simulink model "INS"  (R2018b)
settings: configuration reference "ins_config" (kept outside this file)
values from neighbouring files (symbols this model uses):
  INS_EXPORT = Simulink.Parameter(INS_EXPORT_VALUE)    [ins_model_init.m]
  INS_PARAM = Simulink.Parameter(INS_PARAM_VALUE)    [ins_model_init.m]
undefined symbols (not defined in the file or in its folder): DiscIntNeverNeededParam, INS_CONST, INS_EXPORT_VALUE, Sensor_Meas
libraries: simulink x131, FMT_Model_Lib x48
(part 3 of 6)

== system INS/Data_Fusion/Rotation_Filter/AHRS/Correct/Gyro_Bias_Correction ==
  att_B_correction : Inport
  IMU_Data : Inport  Port=2
  Abs : Abs
  Bus Selector : BusSelector  OutputSignals=acc_B_mPs2
  Compare To Constant : simulink/Logic and Bit Operations/Compare To Constant  relop=<=  const=1  OutDataTypeStr=boolean
  Constant : Constant  Value=INS_CONST.g  OutDataTypeStr=single
  Data Type Conversion : DataTypeConversion  OutDataTypeStr=single
  Demux : Demux  Outputs=3
  Gain1 : Gain  Gain=INS_PARAM.BIAS_G_GAIN
  Gain2 : Gain  Gain=INS_PARAM.BIAS_G_GAIN
  Gain3 : Gain  Gain=0
  MX Product1 : Product  RndMeth=Simplest
  Mux : Mux  Inputs=3
  Saturation2 : Saturate  UpperLimit=0.1/180*pi  LowerLimit=-0.1/180*pi
  Second Order LPF : FMT_Model_Lib/Filter/Second Order LPF  fc=5  zeta=0.707
      settings: SourceProductName=FMT Toolbox
  Subtract : Sum  Inputs=+-
  Vector Modulus : FMT_Model_Lib/Math/Vector Modulus
      settings: SourceProductName=FMT Toolbox
  bias_g_B_correction : Outport
  wires:
  IMU_Data/1 -> Bus Selector/1
  Saturation2/1 -> bias_g_B_correction/1  "bias_g_correction"
  Compare To Constant/1 -> Data Type Conversion/1
  Bus Selector/1 -> Vector Modulus/1  "<acc_B_mPs2>"
  MX Product1/1 -> Second Order LPF/1
  att_B_correction/1 -> MX Product1/1
  Vector Modulus/1 -> Subtract/1
  Mux/1 -> Saturation2/1
  Constant/1 -> Subtract/2
  Subtract/1 -> Abs/1
  Abs/1 -> Compare To Constant/1
  Data Type Conversion/1 -> MX Product1/2
  Second Order LPF/1 -> Demux/1
  Demux/1 -> Gain1/1
  Demux/2 -> Gain2/1
  Demux/3 -> Gain3/1
  Gain1/1 -> Mux/1
  Gain2/1 -> Mux/2
  Gain3/1 -> Mux/3

== system INS/Data_Fusion/Rotation_Filter/AHRS/Update/Attitude_Update ==
  att_reset : Inport
  quat_0 : Inport  Port=2
  att_B_correction : Inport  Port=3
  Constant : Constant  Value=0  OutDataTypeStr=single
  Delay1 : Delay  DelayLength=1  InitialConditionSource=Input port  InitialCondition=[1.0 0 0 0]
      settings: InputPortMap=u0,p4
  Gain1 : Gain  Gain=0.5  OutMin=-450*pi/180  OutMax=450*pi/180  RndMeth=Simplest
  Mux1 : Mux  Inputs=2
  Quaternion Multiply1 : FMT_Model_Lib/Quaternion/Quaternion Multiply
      settings: SourceProductName=FMT Toolbox
  Quaternion Normalize1 : FMT_Model_Lib/Quaternion/Quaternion Normalize
      settings: SourceProductName=FMT Toolbox
  Quaternion To DCM : FMT_Model_Lib/Quaternion/Quaternion To DCM
      settings: SourceProductName=FMT Toolbox
  Sum : Sum  Inputs=++|
  Switch : Switch  Criteria=u2 > Threshold
  Transpose : Math  Operator=transpose  SaturateOnIntegerOverflow=on
  dT : Gain  Gain=INS_CONST.dt  OutDataTypeStr=Inherit: Same as input
  att_quat : Outport
  DCM_OB : Outport  Port=2
  wires:
  att_reset/1 -> Switch/2
  quat_0/1 -> Switch/1, Delay1/2
  att_B_correction/1 -> Mux1/2
  Mux1/1 -> Quaternion Multiply1/2
  Constant/1 -> Mux1/1
  Quaternion To DCM/1 -> Transpose/1
  Transpose/1 -> DCM_OB/1
  Sum/1 -> Quaternion Normalize1/1
  dT/1 -> Sum/1
  Delay1/1 -> Quaternion Multiply1/1, Sum/2
  Quaternion Multiply1/1 -> Gain1/1
  Gain1/1 -> dT/1
  Switch/1 -> Delay1/1
  Quaternion Normalize1/1 -> att_quat/1, Switch/3, Quaternion To DCM/1

== system INS/Data_Fusion/Rotation_Filter/AHRS/Update/Attitude_Update1 ==
  att_reset : Inport
  quat_0 : Inport  Port=2
  att_B_correction : Inport  Port=3
  Constant : Constant  Value=0  OutDataTypeStr=single
  Discrete-Time Integrator : DiscreteIntegrator  ExternalReset=level  InitialConditionSource=external  SampleTime=-1  ICPrevOutput=DiscIntNeverNeededParam  ICPrevScaledInput=DiscIntNeverNeededParam
  Gain2 : Gain  Gain=0.5  OutMin=-450*pi/180  OutMax=450*pi/180  RndMeth=Simplest
  Mux1 : Mux  Inputs=2
  Quaternion Modulus : FMT_Model_Lib/Quaternion/Quaternion Modulus
      settings: SourceProductName=FMT Toolbox
  Quaternion Multiply : FMT_Model_Lib/Quaternion/Quaternion Multiply
      settings: SourceProductName=FMT Toolbox
  Quaternion Normalize : FMT_Model_Lib/Quaternion/Quaternion Normalize
      settings: SourceProductName=FMT Toolbox
  Quaternion To DCM : FMT_Model_Lib/Quaternion/Quaternion To DCM
      settings: SourceProductName=FMT Toolbox
  Transpose : Math  Operator=transpose  SaturateOnIntegerOverflow=on
  att_quat : Outport
  DCM_OB : Outport  Port=2
  wires:
  att_reset/1 -> Discrete-Time Integrator/2
  quat_0/1 -> Discrete-Time Integrator/3
  Gain2/1 -> Discrete-Time Integrator/1
  Quaternion Multiply/1 -> Gain2/1
  att_B_correction/1 -> Mux1/2
  Mux1/1 -> Quaternion Multiply/2
  Constant/1 -> Mux1/1
  Quaternion Normalize/1 -> Quaternion To DCM/1, Quaternion Multiply/1, att_quat/1
  Discrete-Time Integrator/1 -> Quaternion Modulus/1, Quaternion Normalize/1  "dd3"
  Quaternion To DCM/1 -> Transpose/1
  Transpose/1 -> DCM_OB/1
  Quaternion Modulus/1 -> ?  "dd4"

== system INS/Data_Fusion/Rotation_Filter/AHRS/Update/Gyro_Bias_Update ==
  bias_g_correction : Inport
  gyr_B_radPs : Inport  Port=2
  Discrete-Time Integrator2 : DiscreteIntegrator  SampleTime=-1  LimitOutput=on  UpperSaturationLimit=45/180*pi  LowerSaturationLimit=-45/180*pi  ICPrevOutput=DiscIntNeverNeededParam  ICPrevScaledInput=DiscIntNeverNeededParam
  Sum1 : Sum  Inputs=++|
  gyr_B_correction : Outport
  bias_g : Outport  Port=2
  wires:
  bias_g_correction/1 -> Discrete-Time Integrator2/1
  Sum1/1 -> gyr_B_correction/1
  Discrete-Time Integrator2/1 -> Sum1/1, bias_g/1
  gyr_B_radPs/1 -> Sum1/2

== system INS/Data_Fusion/Rotation_Filter/RF_Data_PreProcess/Attitude_Reset/sample_valid ==
  valid : Inport
  Add : Sum  AccumDataTypeStr=uint32
  Data Type Conversion : DataTypeConversion  OutDataTypeStr=uint32
  Delay : Delay  DelayLength=1
  Saturation : Saturate  UpperLimit=10000  LowerLimit=0
  valid_samples : simulink/Logic and Bit Operations/Compare To Constant  relop=>  const=50  OutDataTypeStr=boolean
  imu_valid : Outport
  wires:
  Add/1 -> Saturation/1
  valid_samples/1 -> imu_valid/1
  Delay/1 -> Add/2
  valid/1 -> Data Type Conversion/1
  Data Type Conversion/1 -> Add/1
  Saturation/1 -> valid_samples/1, Delay/1

== system INS/Data_Fusion/Rotation_Filter/RF_Data_PreProcess/Attitude_Reset/sample_valid1 ==
  valid : Inport
  Add : Sum  AccumDataTypeStr=uint32
  Data Type Conversion : DataTypeConversion  OutDataTypeStr=uint32
  Delay : Delay  DelayLength=1
  Saturation : Saturate  UpperLimit=10000  LowerLimit=0
  valid_samples : simulink/Logic and Bit Operations/Compare To Constant  relop=>  const=50  OutDataTypeStr=boolean
  mag_valid : Outport
  wires:
  Add/1 -> Saturation/1
  valid_samples/1 -> mag_valid/1
  Delay/1 -> Add/2
  valid/1 -> Data Type Conversion/1
  Data Type Conversion/1 -> Add/1
  Saturation/1 -> valid_samples/1, Delay/1

== system INS/Data_Fusion/Rotation_Filter/RF_Data_PreProcess/Initial_Attitude/Heading_Vector ==
  Sensor_Data : Inport
  Bus Selector1 : BusSelector  OutputSignals=Mag_Data.mag_norm_B
  Bus Selector2 : BusSelector  OutputSignals=GPS_Data.heading_valid,ExternalPos_Data.height_valid
  Bus Selector3 : BusSelector  OutputSignals=GPS_Data.heading_rad,ExternalPos_Data.psi
  Constant : Constant  Value=[1; 0; 0]  VectorParams1D=off  OutDataTypeStr=single
  Logical Operator : Logic  Operator=OR  AllPortsSameDT=off  OutDataTypeStr=boolean
  Multiply : Product  Multiplication=Matrix(*)
  Psi To DCM : FMT_Model_Lib/Transformation/Psi To DCM
      settings: SourceProductName=FMT Toolbox
  Switch : Switch  Criteria=u2 > Threshold
  Switch1 : Switch  Criteria=u2 > Threshold
  Vector Normalize : FMT_Model_Lib/Math/Vector Normalize
      settings: SourceProductName=FMT Toolbox
  heading_vec : Outport
  wires:
  Psi To DCM/1 -> Multiply/1
  Bus Selector1/1 -> Switch/3  "<mag_norm_B>"
  Switch/1 -> heading_vec/1
  Switch1/1 -> Psi To DCM/1  "<psi>"
  Logical Operator/1 -> Switch/2  "<heading_valid>"
  Sensor_Data/1 -> Bus Selector3/1, Bus Selector2/1, Bus Selector1/1
  Constant/1 -> Multiply/2
  Multiply/1 -> Vector Normalize/1
  Vector Normalize/1 -> Switch/1
  Bus Selector2/2 -> Logical Operator/2  "<height_valid>"
  Bus Selector2/1 -> Switch1/2, Logical Operator/1  "<heading_valid>"
  Bus Selector3/1 -> Switch1/1  "<heading_rad>"
  Bus Selector3/2 -> Switch1/3  "<psi>"

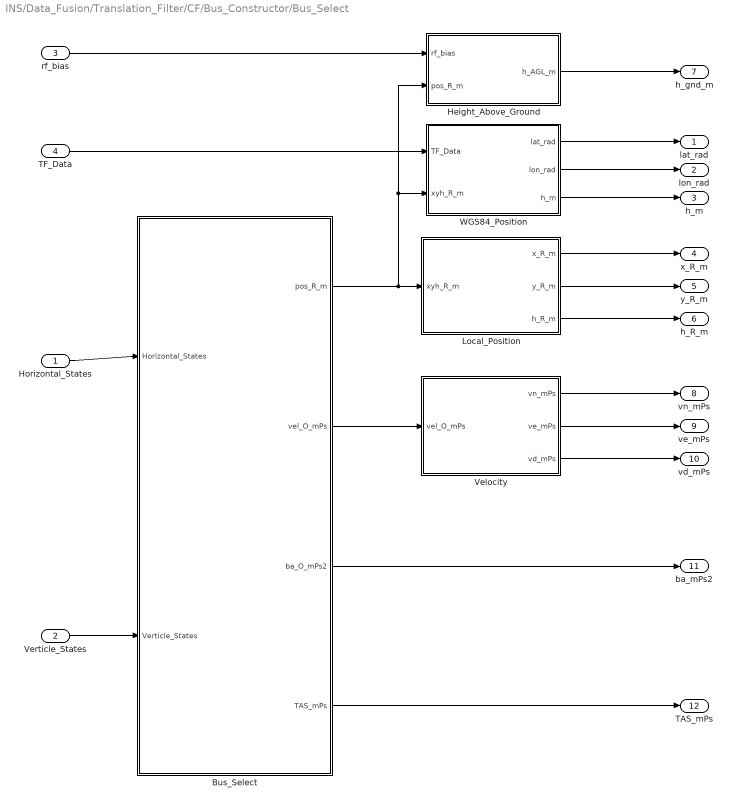
== system INS/Data_Fusion/Translation_Filter/CF/Bus_Constructor/Bus_Select ==
  Horizontal_States : Inport
  Verticle_States : Inport  Port=2
  rf_bias : Inport  Port=3
  TF_Data : Inport  Port=4
  Bus_Select : Subsystem
  Height_Above_Ground : Subsystem
  Local_Position : Subsystem
  Velocity : Subsystem
  WGS84_Position : Subsystem
  lat_rad : Outport
  lon_rad : Outport  Port=2
  h_m : Outport  Port=3
  x_R_m : Outport  Port=4
  y_R_m : Outport  Port=5
  h_R_m : Outport  Port=6
  h_gnd_m : Outport  Port=7
  vn_mPs : Outport  Port=8
  ve_mPs : Outport  Port=9
  vd_mPs : Outport  Port=10
  ba_mPs2 : Outport  Port=11
  TAS_mPs : Outport  Port=12
  wires:
  WGS84_Position/1(lat_rad) -> lat_rad/1
  TF_Data/1 -> WGS84_Position/1(TF_Data)
  WGS84_Position/2(lon_rad) -> lon_rad/1
  WGS84_Position/3(h_m) -> h_m/1
  Local_Position/1(x_R_m) -> x_R_m/1
  Local_Position/2(y_R_m) -> y_R_m/1
  Local_Position/3(h_R_m) -> h_R_m/1
  Bus_Select/1(pos_R_m) -> Local_Position/1(xyh_R_m), Height_Above_Ground/2(pos_R_m), WGS84_Position/2(xyh_R_m)
  Horizontal_States/1 -> Bus_Select/1(Horizontal_States)
  Verticle_States/1 -> Bus_Select/2(Verticle_States)
  Bus_Select/3(ba_O_mPs2) -> ba_mPs2/1
  Height_Above_Ground/1(h_AGL_m) -> h_gnd_m/1
  Bus_Select/2(vel_O_mPs) -> Velocity/1(vel_O_mPs)
  Velocity/1(vn_mPs) -> vn_mPs/1
  Velocity/2(ve_mPs) -> ve_mPs/1
  Velocity/3(vd_mPs) -> vd_mPs/1
  rf_bias/1 -> Height_Above_Ground/1(rf_bias)
  Bus_Select/4(TAS_mPs) -> TAS_mPs/1

== system INS/Data_Fusion/Translation_Filter/CF/Horizontal_Filter/Correct ==
  X_Predict : Inport
  TF_Data : Inport  Port=2
  Airspeed Correct : Subsystem
  ExternalPos Correct : Subsystem
  GPS Correct : Subsystem
  OptFlow Correct : Subsystem
  X_Next : Outport
  wires:
  X_Predict/1 -> OptFlow Correct/1(X_Predict)
  OptFlow Correct/1(X_Next) -> GPS Correct/1(X_Predict)
  TF_Data/1 -> Airspeed Correct/2(TF_Data), ExternalPos Correct/2(TF_Data), GPS Correct/2(TF_Data), OptFlow Correct/2(TF_Data)
  GPS Correct/1(X_Next) -> ExternalPos Correct/1(X_Predict)
  ExternalPos Correct/1(X_Next) -> Airspeed Correct/1(X_Predict)
  Airspeed Correct/1(X_Next) -> X_Next/1

== system INS/Data_Fusion/Translation_Filter/CF/Horizontal_Filter/Predict ==
  X_Prio : Inport
  Rotation_Data : Inport  Port=2
  TF_Data : Inport  Port=3
  Propagate : Subsystem
  Update : Subsystem
  X_Predict : Outport
  wires:
  X_Prio/1 -> Propagate/1(X_prio)
  TF_Data/1 -> Update/2(TF_Data), Propagate/2(TF_Data)
  Propagate/1(X) -> Update/1(X_Prio)
  Rotation_Data/1 -> Update/3(Rotation_Data)
  Update/1(X_Predict) -> X_Predict/1

== system INS/Data_Fusion/Translation_Filter/CF/Verticle_Filter/Correct ==
  X_Predict : Inport
  TF_Data : Inport  Port=2
  Baro_Correct : Subsystem
  ExternalPos_Correct : Subsystem
  GPS_Correct : Subsystem
  Rf_Correct : Subsystem
  X_Next : Outport
  rf_bias : Outport  Port=2
  wires:
  TF_Data/1 -> ExternalPos_Correct/2(TF_Data), Rf_Correct/2(TF_Data), GPS_Correct/2(TF_Data), Baro_Correct/2(TF_Data)
  X_Predict/1 -> Baro_Correct/1(X_Predict)
  Baro_Correct/1(X_Next) -> GPS_Correct/1(X_Predict)
  GPS_Correct/1(X_Next) -> Rf_Correct/1(X_Predict)
  ExternalPos_Correct/1(X_Next) -> X_Next/1
  Rf_Correct/1(X_Next) -> ExternalPos_Correct/1(X_Predict)
  Rf_Correct/2(rf_bias) -> rf_bias/1

== system INS/Data_Fusion/Translation_Filter/CF/Verticle_Filter/Predict ==
  X_Prio : Inport
  Rotation_Data : Inport  Port=2
  TF_Data : Inport  Port=3
  Propagate : Subsystem
  Update : Subsystem
  X_Predict : Outport
  wires:
  X_Prio/1 -> Propagate/1(X_Prio)
  TF_Data/1 -> Update/2(TF_Data), Propagate/2(TF_Data)
  Propagate/1(X) -> Update/1(X_Prio)
  Rotation_Data/1 -> Update/3(Rotation_Data)
  Update/1(X_Predict) -> X_Predict/1

== system INS/Data_Fusion/Translation_Filter/TF_Data_PreProcess/Sensor_Process/Sensor_Select ==
  Sensor_Status : Inport
  Bus Creator : BusCreator  Inputs=2
  Horizontal_Sensor_Select : Subsystem
  Vertical_Sensor_Select : Subsystem
  Sensor_Select : Outport
  wires:
  Sensor_Status/1 -> Vertical_Sensor_Select/1(Sensor_Status), Horizontal_Sensor_Select/1(Sensor_Status)
  Bus Creator/1 -> Sensor_Select/1
  Horizontal_Sensor_Select/1(horizon_select) -> Bus Creator/1  "horizon_select"
  Vertical_Sensor_Select/1(vert_select) -> Bus Creator/2  "vert_select"

== system INS/Data_Fusion/Translation_Filter/TF_Data_PreProcess/Sensor_Process/TF_Sensor_Measures ==
  Sensor_Data : Inport
  Rotation_Data : Inport  Port=2
  Airspeed_Meas : Subsystem
  Barometer_Meas : Subsystem
  Bus Creator : BusCreator  Inputs=6
  ExternalPos_Meas : Subsystem
  GPS_Meas : Subsystem
  OpticalFlow_Meas : Subsystem
  Rangefinder_Meas : Subsystem
  Sensor_Meas : Outport
  wires:
  Bus Creator/1 -> Sensor_Meas/1
  Sensor_Data/1 -> Airspeed_Meas/1(Sensor_Data), ExternalPos_Meas/1(Sensor_Data), OpticalFlow_Meas/1(Sensor_Data), Rangefinder_Meas/1(Sensor_Data), Barometer_Meas/1(Sensor_Data), GPS_Meas/1(Sensor_Data)
  GPS_Meas/1(GPS_Meas) -> Bus Creator/1  "GPS_Meas"
  Barometer_Meas/1(Baro_Meas) -> Bus Creator/2  "Baro_Meas"
  Rangefinder_Meas/1(Rf_Meas) -> Bus Creator/3  "Rf_Meas"
  OpticalFlow_Meas/1(OptFlow_Meas) -> Bus Creator/4  "OptFlow_Meas"
  Rotation_Data/1 -> OpticalFlow_Meas/2(Rotation_Data), ExternalPos_Meas/2(Rotation_Data)
  ExternalPos_Meas/1(ExtPos_Meas) -> Bus Creator/5  "ExtPos_Meas"
  Airspeed_Meas/1(Airspeed_Meas) -> Bus Creator/6  "Airspeed_Meas"

== system INS/Data_Fusion/Translation_Filter/TF_Data_PreProcess/Sensor_Process/TF_Sensor_Status ==
  Sensor_Data : Inport
  Rotation_Data : Inport  Port=2
  Airspeed_Status : Subsystem
  Barometer_Status : Subsystem
  Bus Creator : BusCreator  Inputs=6
  ExternalPos_Status : Subsystem
  GPS_Status : Subsystem
  OpticalFlow_Status : Subsystem
  Rangefinder_Status : Subsystem
  Sensor_Status : Outport
  wires:
  Bus Creator/1 -> Sensor_Status/1
  Sensor_Data/1 -> Airspeed_Status/1(Sensor_Data), ExternalPos_Status/1(Sensor_Data), OpticalFlow_Status/1(Sensor_Data), Rangefinder_Status/1(Sensor_Data), Barometer_Status/1(Sensor_Data), GPS_Status/1(Sensor_Data)
  GPS_Status/1(GPS_Status) -> Bus Creator/1  "GPS_Status"
  Barometer_Status/1(Baro_Status) -> Bus Creator/2  "Baro_Status"
  Rangefinder_Status/1(Rf_Status) -> Bus Creator/3  "Rf_Status"
  OpticalFlow_Status/1(OptFlow_Status) -> Bus Creator/4  "OptFlow_Status"
  ExternalPos_Status/1(ExtPos_Status) -> Bus Creator/5  "ExternalPos_Status"
  Rotation_Data/1 -> GPS_Status/2(Rotation_Data)
  Airspeed_Status/1(Airspeed_Status) -> Bus Creator/6  "Airspeed_Status"

== system INS/Data_Fusion/Translation_Filter/TF_Data_PreProcess/TF_Data_Post_Process/GPS_OFFSET_Compensation ==
  TF_Data : Inport
  Rotation_Data : Inport  Port=2
  Demux : Demux  Outputs=3
  Demux1 : Demux  Outputs=3
  GPS_POS_Compensation : Subsystem
  GPS_VEL_Compensation : Subsystem
  GPS_X_PFFSET : Constant  Value=INS_PARAM.GPS_X_OFFSET
  GPS_Y_OFFSET : Constant  Value=INS_PARAM.GPS_Y_OFFSET
  GPS_Z_OFFSET : Constant  Value=INS_PARAM.GPS_Z_OFFSET
  Gain : Gain  Gain=-1
  Mux : Mux  Inputs=3
  x_m : Outport
  y_m : Outport  Port=2
  h_m : Outport  Port=3
  vn_mPs : Outport  Port=4
  ve_mPs : Outport  Port=5
  vd_mPs : Outport  Port=6
  wires:
  Demux/1 -> x_m/1
  Demux/2 -> y_m/1
  Demux/3 -> Gain/1
  Rotation_Data/1 -> GPS_VEL_Compensation/1(Rotation_Data), GPS_POS_Compensation/1(Rotation_Data)
  TF_Data/1 -> GPS_VEL_Compensation/2(TF_Data), GPS_POS_Compensation/2(TF_Data)
  Gain/1 -> h_m/1
  GPS_POS_Compensation/1(pos_O_m) -> Demux/1
  GPS_Z_OFFSET/1 -> Mux/3
  GPS_Y_OFFSET/1 -> Mux/2
  GPS_X_PFFSET/1 -> Mux/1
  Mux/1 -> GPS_POS_Compensation/3(GPS_Offset), GPS_VEL_Compensation/3(GPS_Offset)
  GPS_VEL_Compensation/1(vel_O_mPs) -> Demux1/1
  Demux1/1 -> vn_mPs/1
  Demux1/2 -> ve_mPs/1
  Demux1/3 -> vd_mPs/1

== system INS/Data_Fusion/Translation_Filter/TF_Data_PreProcess/Transfer_Filter_Control/Filter_Reset ==
  note: Height_Reset
  note: Position_Reset
  Sensor_Valid : Inport
  Bus Selector : BusSelector  OutputSignals=xy_R_valid
  Bus Selector1 : BusSelector  OutputSignals=h_R_valid
  Detect Rise Positive : simulink/Logic and Bit Operations/Detect Rise Positive  vinit=0  OutDataTypeStr=boolean
  Detect Rise Positive1 : simulink/Logic and Bit Operations/Detect Rise Positive  vinit=0  OutDataTypeStr=boolean
  pos_reset : Outport
  height_reset : Outport  Port=2
  wires:
  Bus Selector/1 -> Detect Rise Positive/1  "<xy_R_valid>"
  Bus Selector1/1 -> Detect Rise Positive1/1  "<h_R_valid>"
  Sensor_Valid/1 -> Bus Selector1/1, Bus Selector/1
  Detect Rise Positive/1 -> pos_reset/1
  Detect Rise Positive1/1 -> height_reset/1

== system INS/Data_Fusion/Translation_Filter/TF_Data_PreProcess/Transfer_Filter_Control/Sensor_Valid ==
  Sensor_Enable : Inport
  Bus Creator : BusCreator  Inputs=6
  Horizon_Sensor_Valid : Subsystem
  Vertical_Sensor_Valid : Subsystem
  Sensor_Valid : Outport
  wires:
  Horizon_Sensor_Valid/1(lon_lat_valid) -> Bus Creator/1  "lon_lat_valid"
  Horizon_Sensor_Valid/2(xy_R_valid) -> Bus Creator/2  "xy_R_valid"
  Vertical_Sensor_Valid/1(altitude_valid) -> Bus Creator/4  "altitude_valid"
  Vertical_Sensor_Valid/2(h_R_valid) -> Bus Creator/5  "h_R_valid"
  Bus Creator/1 -> Sensor_Valid/1
  Sensor_Enable/1 -> Horizon_Sensor_Valid/1(Sensor_Enable), Vertical_Sensor_Valid/1(Sensor_Enable)
  Vertical_Sensor_Valid/3(h_AGL_valid) -> Bus Creator/6  "h_AGL_valid"
  Horizon_Sensor_Valid/3(airspeed_valid) -> Bus Creator/3  "airspeed_valid"

== system INS/Data_Fusion/Translation_Filter/TF_Data_PreProcess/Transfer_Filter_Control/WGS84_Reference ==
  Sensor_Valid : Inport
  Translation_Data : Inport  Port=2
  Sensor_Meas : Inport  Port=3
  Bus_Constructor : Subsystem
  Bus_Select : Subsystem
  Height_Ref : Subsystem
  Position_Ref : Subsystem
  WGS84_Ref : Outport
  wires:
  Bus_Select/2(WGS84_position) -> Position_Ref/4(WGS84_position), Height_Ref/4(WGS84_position)
  Translation_Data/1 -> Height_Ref/1(Translation_Data), Position_Ref/1(Translation_Data)
  Sensor_Valid/1 -> Height_Ref/2(Sensor_Valid), Position_Ref/2(Sensor_Valid)
  Bus_Select/1(WGS84_derivatives) -> Height_Ref/3(WGS84_derivatives), Position_Ref/3(WGS84_derivatives)
  Position_Ref/1(WGS84_pos_ref) -> Bus_Constructor/1(WGS84_pos_ref)
  Position_Ref/2(WGS84_dpos_ref) -> Bus_Constructor/2(WGS84_dpos_ref)
  Height_Ref/1(WGS84_hgt_ref) -> Bus_Constructor/3(WGS84_hgt_ref)
  Height_Ref/2(WGS84_dhgt_ref) -> Bus_Constructor/4(WGS84_dhgt_ref)
  Bus_Constructor/1(WGS84_Ref) -> WGS84_Ref/1
  Sensor_Meas/1 -> Bus_Select/1(Sensor_Meas)

== system INS/Sensor_PreProcess/GPS_PreProcess/Status_Quality/GPS_Status/Ready ==
  valid : Inport
  Saturation : Saturate  UpperLimit=1e4  LowerLimit=0
  Sum : Sum  Inputs=|++  OutDataTypeStr=int32
  Unit Delay : UnitDelay  SampleTime=-1
  valid_samples : simulink/Logic and Bit Operations/Compare To Constant  relop=>=  const=1000  OutDataTypeStr=boolean
  ready : Outport
  wires:
  valid_samples/1 -> ready/1
  Sum/1 -> Saturation/1
  Unit Delay/1 -> valid_samples/1, Sum/2
  Saturation/1 -> Unit Delay/1
  valid/1 -> Sum/1

== system INS/Sensor_PreProcess/MAG_PreProcess/Mag_Data_Process/Mag_Quality_Estimate/Mag_Quality ==
  nominal_inc_deg : Inport
  mag_normalized_O : Inport  Port=2
  Inclination_Quality_Estimate : Subsystem
  Intensity_Quality_Estimate : Subsystem
  MinMax : MinMax  Inputs=2
  Saturation : Saturate  UpperLimit=1  LowerLimit=0.1
  Second Order LPF : FMT_Model_Lib/Filter/Second Order LPF  fc=5  zeta=0.707
      settings: SourceProductName=FMT Toolbox
  mag_quality : Outport
  wires:
  Intensity_Quality_Estimate/1(intensity_quality) -> MinMax/2  "mag_int_quality"
  nominal_inc_deg/1 -> Inclination_Quality_Estimate/1(nominal_inc_deg)
  Inclination_Quality_Estimate/1(inclination_quality) -> MinMax/1  "mag_inc_quality"
  mag_normalized_O/1 -> Inclination_Quality_Estimate/2(mag_normalized_O), Intensity_Quality_Estimate/1(mag_normalized_O)
  MinMax/1 -> Second Order LPF/1
  Second Order LPF/1 -> Saturation/1
  Saturation/1 -> mag_quality/1

== system INS/Sensor_PreProcess/MAG_PreProcess/Mag_Data_Process/WMM_Compensation/safe_divide ==
  u1 : Inport
  u2 : Inport  Port=2
  Constant1 : Constant  VectorParams1D=off  OutDataTypeStr=single
  Divide1 : Product  Inputs=*/
  MinMax : MinMax  Function=max  Inputs=2
  y : Outport
  wires:
  MinMax/1 -> Divide1/2
  Constant1/1 -> MinMax/1
  Divide1/1 -> y/1
  u2/1 -> MinMax/2
  u1/1 -> Divide1/1

== system INS/Data_Fusion/Rotation_Filter/AHRS/Correct/Attitude_Correction/Attitude_Correct ==
  Rotation_Data : Inport
  Sensor_Data : Inport  Port=2
  RF_Data : Inport  Port=3
  Acc_Correct : Subsystem
  Acc_Estimator : Subsystem
  att_corr_O : Outport
  wires:
  Acc_Estimator/3(acc_est_O_mPs2) -> Acc_Correct/3(acc_est_O_mPs2)  "acc_est_O_mPs2"
  Sensor_Data/1 -> Acc_Estimator/2(Sensor_Data)
  Rotation_Data/1 -> Acc_Estimator/3(Rotation_Data)
  Acc_Correct/1(att_correct) -> att_corr_O/1
  Acc_Estimator/1(acc_meas_valid) -> Acc_Correct/1(acc_meas_valid)  "acc_meas_valid"
  Acc_Estimator/2(acc_meas_O_mPs2) -> Acc_Correct/2(acc_meas_O_mPs2)  "acc_meas_O_mPs2"
  RF_Data/1 -> Acc_Estimator/1(RF_Data)

== system INS/Data_Fusion/Rotation_Filter/AHRS/Correct/Attitude_Correction/ExternalPsi_Correct ==
  RF_Data : Inport
  Rotation_Data : Inport  Port=2
  Sensor_Data : Inport  Port=3
  Bias_Estimation : Subsystem
  Bus Selector : BusSelector  OutputSignals=ExternalPos_Data.psi
  Bus Selector1 : BusSelector  OutputSignals=ext_psi_enable
  Bus Selector2 : BusSelector  OutputSignals=psi_rad
  Detect Increase : simulink/Logic and Bit Operations/Detect Increase  vinit=0.0  OutDataTypeStr=boolean
  Gain : Gain  Gain=[0; 0; 1]
  Multiply : Product
  Sum : Sum  Inputs=++-
  psi_err_saturation : Subsystem
  att_corr_O : Outport
  wires:
  Rotation_Data/1 -> Bus Selector2/1
  Gain/1 -> Multiply/2
  psi_err_saturation/1(psi_err_rad) -> Gain/1
  Sensor_Data/1 -> Bus Selector/1
  Sum/1 -> psi_err_saturation/1(psi_err_in)
  Bus Selector1/1 -> Detect Increase/1, Multiply/1  "<ext_psi_enable>"
  Multiply/1 -> att_corr_O/1
  Bus Selector/1 -> Sum/2, Bias_Estimation/2(psi_meas)  "<psi>"
  Bus Selector2/1 -> Bias_Estimation/3(psi_est), Sum/3  "<psi_rad>"
  RF_Data/1 -> Bus Selector1/1
  Detect Increase/1 -> Bias_Estimation/1(bias_update)
  Bias_Estimation/1(bias) -> Sum/1  "ext_psi_bias"

== system INS/Data_Fusion/Rotation_Filter/AHRS/Correct/Attitude_Correction/GPS_Heading_Correct ==
  RF_Data : Inport
  Rotation_Data : Inport  Port=2
  Sensor_Data : Inport  Port=3
  Bus Selector : BusSelector  OutputSignals=GPS_Data.heading_rad
  Bus Selector1 : BusSelector  OutputSignals=gps_psi_enable
  Bus Selector2 : BusSelector  OutputSignals=psi_rad
  Gain : Gain  Gain=[0; 0; 1]
  Multiply : Product
  Sum : Sum  Inputs=|+-
  psi_err_saturation : Subsystem
  att_corr_O : Outport
  wires:
  Rotation_Data/1 -> Bus Selector2/1
  Gain/1 -> Multiply/2
  psi_err_saturation/1(psi_err_rad) -> Gain/1
  Sensor_Data/1 -> Bus Selector/1
  Sum/1 -> psi_err_saturation/1(psi_err_in)
  Multiply/1 -> att_corr_O/1
  Bus Selector/1 -> Sum/1  "<heading_rad>"
  Bus Selector2/1 -> Sum/2  "<psi_rad>"
  Bus Selector1/1 -> Multiply/1  "<gps_psi_enable>"
  RF_Data/1 -> Bus Selector1/1

== system INS/Data_Fusion/Rotation_Filter/AHRS/Correct/Attitude_Correction/Mag_Correct ==
  Rotation_Data : Inport
  Sensor_Data : Inport  Port=2
  RF_Data : Inport  Port=3
  Translation_Data : Inport  Port=4
  Bus Selector : BusSelector  OutputSignals=psi_rad
  Bus Selector1 : BusSelector  OutputSignals=Mag_Data.mag_norm_B
  Constant : Constant  Value=[0 0]  OutDataTypeStr=single
  Gain3 : Gain  Gain=INS_PARAM.MAG_GAIN
  Mag_Control : Subsystem
  Mag_Measure : Subsystem
  Multiply : Product
  Mux : Mux  Inputs=2
  Sum : Sum  Inputs=+-|
  psi_err_saturation : Subsystem
  mag_corr_O : Outport
  wires:
  Sensor_Data/1 -> Bus Selector1/1, Mag_Control/3(Sensor_Data)
  Rotation_Data/1 -> Bus Selector/1, Mag_Measure/3(Rotation_Data), Mag_Control/2(Rotation_Data)
  Sum/1 -> psi_err_saturation/1(psi_err_in)
  RF_Data/1 -> Mag_Control/1(RF_Data)
  Multiply/1 -> mag_corr_O/1
  Bus Selector1/1 -> Mag_Measure/2(mag_norm_B)  "<mag_norm_B>"
  Bus Selector/1 -> Sum/2  "<psi_rad>"
  Mag_Measure/1(psi_meas) -> Sum/1
  psi_err_saturation/1(psi_err_rad) -> Gain3/1
  Gain3/1 -> Mux/2
  Constant/1 -> Mux/1
  Mux/1 -> Multiply/2
  Mag_Control/2(mag_bias_update) -> Mag_Measure/1(bias_update)
  Mag_Control/1(use_mag) -> Multiply/1
  Translation_Data/1 -> Mag_Control/4(Translation_Data)

== system INS/Data_Fusion/Translation_Filter/CF/Bus_Constructor/Bus_Select/Bus_Select ==
  Horizontal_States : Inport
  Verticle_States : Inport  Port=2
  Mux : Mux  Inputs=2
  Mux1 : Mux  Inputs=2
  Mux2 : Mux  Inputs=2
  Mux3 : Mux  Inputs=1
  Selector : Selector  InputPortWidth=7  IndexOptions=Index vector (dialog)  Indices=[1 2]  OutputSizes=1
  Selector1 : Selector  InputPortWidth=3  IndexOptions=Index vector (dialog)  Indices=[1]  OutputSizes=1
  Selector2 : Selector  InputPortWidth=7  IndexOptions=Index vector (dialog)  Indices=[3 4]  OutputSizes=1
  Selector3 : Selector  InputPortWidth=3  IndexOptions=Index vector (dialog)  Indices=[2]  OutputSizes=1
  Selector4 : Selector  InputPortWidth=7  IndexOptions=Index vector (dialog)  Indices=[5 6]  OutputSizes=1
  Selector5 : Selector  InputPortWidth=3  IndexOptions=Index vector (dialog)  Indices=[3]  OutputSizes=1
  Selector6 : Selector  InputPortWidth=7  IndexOptions=Index vector (dialog)  Indices=7  OutputSizes=1
  pos_R_m : Outport
  vel_O_mPs : Outport  Port=2
  ba_O_mPs2 : Outport  Port=3
  TAS_mPs : Outport  Port=4
  wires:
  Selector5/1 -> Mux2/2
  Horizontal_States/1 -> Selector6/1, Selector4/1, Selector2/1, Selector/1
  Selector4/1 -> Mux2/1
  Selector2/1 -> Mux1/1
  Selector1/1 -> Mux/2
  Selector/1 -> Mux/1
  Selector3/1 -> Mux1/2
  Mux1/1 -> vel_O_mPs/1
  Verticle_States/1 -> Selector5/1, Selector3/1, Selector1/1
  Mux/1 -> pos_R_m/1
  Mux2/1 -> ba_O_mPs2/1
  Selector6/1 -> Mux3/1
  Mux3/1 -> TAS_mPs/1

== system INS/Data_Fusion/Translation_Filter/CF/Bus_Constructor/Bus_Select/Height_Above_Ground ==
  rf_bias : Inport
  pos_R_m : Inport  Port=2
  Selector : Selector  InputPortWidth=3  IndexOptions=Index vector (dialog)  Indices=3  OutputSizes=1
  Sum : Sum  Inputs=|-+
  h_AGL_m : Outport
  wires:
  rf_bias/1 -> Sum/1
  pos_R_m/1 -> Selector/1
  Sum/1 -> h_AGL_m/1
  Selector/1 -> Sum/2

== system INS/Data_Fusion/Translation_Filter/CF/Bus_Constructor/Bus_Select/Local_Position ==
  xyh_R_m : Inport
  Demux : Demux  Outputs=3
  x_R_m : Outport
  y_R_m : Outport  Port=2
  h_R_m : Outport  Port=3
  wires:
  Demux/2 -> y_R_m/1
  Demux/1 -> x_R_m/1
  Demux/3 -> h_R_m/1
  xyh_R_m/1 -> Demux/1

== system INS/Data_Fusion/Translation_Filter/CF/Bus_Constructor/Bus_Select/Velocity ==
  vel_O_mPs : Inport
  Demux : Demux  Outputs=3
  vn_mPs : Outport
  ve_mPs : Outport  Port=2
  vd_mPs : Outport  Port=3
  wires:
  Demux/3 -> vd_mPs/1
  Demux/1 -> vn_mPs/1
  Demux/2 -> ve_mPs/1
  vel_O_mPs/1 -> Demux/1

== system INS/Data_Fusion/Translation_Filter/CF/Bus_Constructor/Bus_Select/WGS84_Position ==
  TF_Data : Inport
  xyh_R_m : Inport  Port=2
  Bus Selector2 : BusSelector  OutputSignals=Sensor_Status.GPS_Status.gps_vaid
  Data Type Conversion2 : DataTypeConversion  OutDataTypeStr=double
  Demux2 : Demux  Outputs=3
  Multiply : Product
  WGS84_Position : Subsystem
  lat_rad : Outport
  lon_rad : Outport  Port=2
  h_m : Outport  Port=3
  wires:
  WGS84_Position/1(WGS84_pos) -> Multiply/2
  TF_Data/1 -> Bus Selector2/1, WGS84_Position/2(TF_Data)
  Bus Selector2/1 -> Data Type Conversion2/1  "<gps_vaid>"
  Data Type Conversion2/1 -> Multiply/1
  Multiply/1 -> Demux2/1
  xyh_R_m/1 -> WGS84_Position/1(xyh_R_m)
  Demux2/1 -> lat_rad/1  "lat_rad"
  Demux2/2 -> lon_rad/1  "lon_rad"
  Demux2/3 -> h_m/1  "h_m"

== system INS/Data_Fusion/Translation_Filter/CF/Horizontal_Filter/Correct/Airspeed Correct ==
  X_Predict : Inport
  TF_Data : Inport  Port=2
  Airspeed_Correct : Subsystem
  Bus Selector : BusSelector  OutputSignals=Sensor_Enable.horizon_select.airspeed_enable
  Switch : Switch  Criteria=u2 > Threshold
  X_Next : Outport
  wires:
  TF_Data/1 -> Bus Selector/1, Airspeed_Correct/1(TF_Data)
  Bus Selector/1 -> Switch/2, Airspeed_Correct/Enable  "<airspeed_enable>"
  X_Predict/1 -> Switch/3, Airspeed_Correct/2(X_Predict)
  Switch/1 -> X_Next/1
  Airspeed_Correct/1(X_Next) -> Switch/1

== system INS/Data_Fusion/Translation_Filter/CF/Horizontal_Filter/Correct/ExternalPos Correct ==
  X_Predict : Inport
  TF_Data : Inport  Port=2
  Bus Selector : BusSelector  OutputSignals=Sensor_Enable.horizon_select.extpos_enable
  ExternalPos_Correct : Subsystem
  Switch : Switch  Criteria=u2 > Threshold
  X_Next : Outport
  wires:
  ExternalPos_Correct/1(X_Next) -> Switch/1
  Switch/1 -> X_Next/1
  X_Predict/1 -> ExternalPos_Correct/2(X_Predict), Switch/3
  Bus Selector/1 -> ExternalPos_Correct/Enable, Switch/2  "<extpos_enable>"
  TF_Data/1 -> ExternalPos_Correct/1(TF_Data), Bus Selector/1

== system INS/Data_Fusion/Translation_Filter/CF/Horizontal_Filter/Correct/GPS Correct ==
  X_Predict : Inport
  TF_Data : Inport  Port=2
  Bus Selector : BusSelector  OutputSignals=Sensor_Enable.horizon_select.gps_enable
  GPS_Correct : Subsystem
  Switch : Switch  Criteria=u2 > Threshold
  X_Next : Outport
  wires:
  GPS_Correct/1(X_Next) -> Switch/1
  Switch/1 -> X_Next/1
  X_Predict/1 -> GPS_Correct/2(X_Predict), Switch/3
  Bus Selector/1 -> GPS_Correct/Enable, Switch/2  "<gps_enable>"
  TF_Data/1 -> GPS_Correct/1(TF_Data), Bus Selector/1

== system INS/Data_Fusion/Translation_Filter/CF/Horizontal_Filter/Correct/OptFlow Correct ==
  X_Predict : Inport
  TF_Data : Inport  Port=2
  Bus Selector : BusSelector  OutputSignals=Sensor_Enable.horizon_select.optflow_enable
  OptFlow_Correct : Subsystem
  Switch : Switch  Criteria=u2 > Threshold
  X_Next : Outport
  wires:
  OptFlow_Correct/1(X_Next) -> Switch/1
  Switch/1 -> X_Next/1
  X_Predict/1 -> OptFlow_Correct/2(X_Predict), Switch/3
  Bus Selector/1 -> OptFlow_Correct/Enable, Switch/2  "<optflow_enable>"
  TF_Data/1 -> OptFlow_Correct/1(TF_Data), Bus Selector/1

== system INS/Data_Fusion/Translation_Filter/CF/Horizontal_Filter/Predict/Propagate ==
  X_prio : Inport
  TF_Data : Inport  Port=2
  Bus Selector : BusSelector  OutputSignals=TF_Control.pos_reset
  Delay : Delay  DelayLength=1
  States_Init : Subsystem
  Switch : Switch  Criteria=u2 > Threshold
  X : Outport
  wires:
  Delay/1 -> Switch/3
  States_Init/1(X_0) -> Switch/1
  Switch/1 -> X/1  "States_X"
  Bus Selector/1 -> Switch/2  "<pos_reset>"
  TF_Data/1 -> Bus Selector/1, States_Init/1(TF_Data)
  X_prio/1 -> Delay/1

== system INS/Data_Fusion/Translation_Filter/CF/Horizontal_Filter/Predict/Update ==
  note: TODO: Subtract acc bias
  X_Prio : Inport
  TF_Data : Inport  Port=2
  Rotation_Data : Inport  Port=3
  Add : Sum  Inputs=-+
  Assignment : Assignment  DiagnosticForDimensions=Warning  IndexOptions=Index vector (dialog)  Indices=[3:6]  OutputSizes=1
  Bus Selector : BusSelector  OutputSignals=TF_Control.sensor_valid.xy_R_valid
  Bus Selector2 : BusSelector  OutputSignals=M_OB,acc_B_mPs2
  Constant : Constant  Value=[0;0]  OutDataTypeStr=single
  Constant1 : Constant  Value=[0;0;0;0]  VectorParams1D=off  OutDataTypeStr=single
  Gain : Gain  Gain=INS_CONST.dt  OutDataTypeStr=Inherit: Same as input
  Multiply : Product  Multiplication=Matrix(*)
  Mux : Mux
  Reshape : Reshape  OutputDimensionality=Column vector (2-D)  OutputDimensions=[7,1]
  Selector : Selector  InputPortWidth=3  IndexOptions=Index vector (dialog)  Indices=[1 2]  OutputSizes=1
  Selector1 : Selector  InputPortWidth=7  IndexOptions=Index vector (dialog)  Indices=[3 4]  OutputSizes=1
  Selector2 : Selector  InputPortWidth=7  IndexOptions=Index vector (dialog)  Indices=[5 6]  OutputSizes=1
  Selector3 : Selector  InputPortWidth=3  IndexOptions=Index vector (dialog)  Indices=1  OutputSizes=1
  Sum : Sum  Inputs=++|
  Switch : Switch  Criteria=u2 > Threshold
  X_Predict : Outport
  wires:
  Rotation_Data/1 -> Bus Selector2/1
  Bus Selector2/1 -> Multiply/1  "<M_OB>"
  Multiply/1 -> Selector/1  "acc_O"
  Bus Selector2/2 -> Selector3/1, Multiply/2  "<acc_B_mPs2>"
  X_Prio/1 -> Selector1/1, Sum/1, Selector2/1
  Selector/1 -> Add/2
  Constant/1 -> Mux/3
  Mux/1 -> Reshape/1
  Reshape/1 -> Gain/1
  Sum/1 -> Assignment/1, Switch/1
  Selector2/1 -> Add/1
  Selector3/1 -> Mux/4
  TF_Data/1 -> Bus Selector/1
  Selector1/1 -> Mux/1
  Add/1 -> Mux/2
  Bus Selector/1 -> Switch/2  "<xy_R_valid>"
  Assignment/1 -> Switch/3
  Switch/1 -> X_Predict/1
  Constant1/1 -> Assignment/2
  Gain/1 -> Sum/2

== system INS/Data_Fusion/Translation_Filter/CF/Verticle_Filter/Correct/Baro_Correct ==
  X_Predict : Inport
  TF_Data : Inport  Port=2
  Baro_Correct : Subsystem
  Bus Selector : BusSelector  OutputSignals=Sensor_Enable.vert_select.baro_enable
  Switch : Switch  Criteria=u2 > Threshold
  X_Next : Outport
  wires:
  Switch/1 -> X_Next/1
  Bus Selector/1 -> Baro_Correct/Enable, Switch/2  "<baro_enable>"
  TF_Data/1 -> Baro_Correct/1(TF_Data), Bus Selector/1
  Baro_Correct/1(X_Next) -> Switch/1
  X_Predict/1 -> Baro_Correct/2(X_Predict), Switch/3

== system INS/Data_Fusion/Translation_Filter/CF/Verticle_Filter/Correct/ExternalPos_Correct ==
  X_Predict : Inport
  TF_Data : Inport  Port=2
  Bus Selector : BusSelector  OutputSignals=Sensor_Enable.vert_select.extpos_enable
  ExternalPos_Correct : Subsystem
  Switch : Switch  Criteria=u2 > Threshold
  X_Next : Outport
  wires:
  Switch/1 -> X_Next/1
  Bus Selector/1 -> ExternalPos_Correct/Enable, Switch/2  "<extpos_enable>"
  TF_Data/1 -> ExternalPos_Correct/1(TF_Data), Bus Selector/1
  ExternalPos_Correct/1(X_Next) -> Switch/1
  X_Predict/1 -> ExternalPos_Correct/2(X_Predict), Switch/3

== system INS/Data_Fusion/Translation_Filter/CF/Verticle_Filter/Correct/GPS_Correct ==
  X_Predict : Inport
  TF_Data : Inport  Port=2
  Bus Selector : BusSelector  OutputSignals=Sensor_Enable.vert_select.gps_enable
  GPS_Correct : Subsystem
  Switch : Switch  Criteria=u2 > Threshold
  X_Next : Outport
  wires:
  Switch/1 -> X_Next/1
  Bus Selector/1 -> GPS_Correct/Enable, Switch/2  "<gps_enable>"
  TF_Data/1 -> GPS_Correct/1(TF_Data), Bus Selector/1
  GPS_Correct/1(X_Next) -> Switch/1
  X_Predict/1 -> GPS_Correct/2(X_Predict), Switch/3

== system INS/Data_Fusion/Translation_Filter/CF/Verticle_Filter/Correct/Rf_Correct ==
  X_Predict : Inport
  TF_Data : Inport  Port=2
  Bus Selector : BusSelector  OutputSignals=Sensor_Enable.vert_select.rf_enable
  Rangefinder_Correct : Subsystem
  Switch : Switch  Criteria=u2 > Threshold
  X_Next : Outport
  rf_bias : Outport  Port=2
  wires:
  Switch/1 -> X_Next/1
  Bus Selector/1 -> Rangefinder_Correct/Enable, Switch/2  "<rf_enable>"
  TF_Data/1 -> Rangefinder_Correct/1(TF_Data), Bus Selector/1
  Rangefinder_Correct/1(X_Next) -> Switch/1
  X_Predict/1 -> Rangefinder_Correct/2(X_Predict), Switch/3
  Rangefinder_Correct/2(rf_bias) -> rf_bias/1

== system INS/Data_Fusion/Translation_Filter/CF/Verticle_Filter/Predict/Propagate ==
  X_Prio : Inport
  TF_Data : Inport  Port=2
  Bus Selector : BusSelector  OutputSignals=TF_Control.height_reset
  Delay : Delay  DelayLength=1
  States_Init : Subsystem
  Switch : Switch  Criteria=u2 > Threshold
  X : Outport
  wires:
  X_Prio/1 -> Delay/1
  TF_Data/1 -> States_Init/1(TF_Data), Bus Selector/1
  Bus Selector/1 -> Switch/2  "<height_reset>"
  Switch/1 -> X/1
  States_Init/1(X_0) -> Switch/1
  Delay/1 -> Switch/3

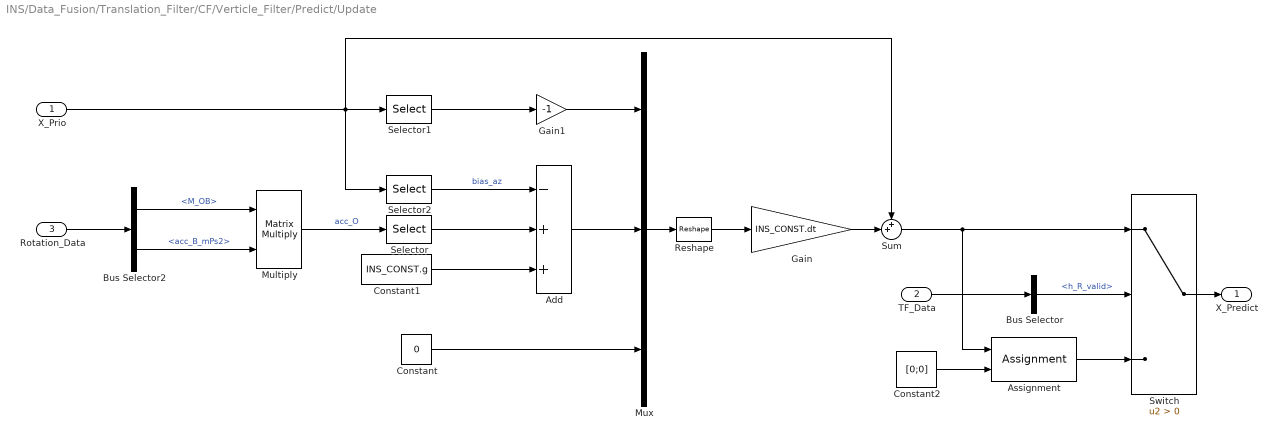
== system INS/Data_Fusion/Translation_Filter/CF/Verticle_Filter/Predict/Update ==
  X_Prio : Inport
  TF_Data : Inport  Port=2
  Rotation_Data : Inport  Port=3
  Add : Sum  Inputs=-++
  Assignment : Assignment  DiagnosticForDimensions=Warning  IndexOptions=Index vector (dialog)  Indices=[2:3]  OutputSizes=1
  Bus Selector : BusSelector  OutputSignals=TF_Control.sensor_valid.h_R_valid
  Bus Selector2 : BusSelector  OutputSignals=M_OB,acc_B_mPs2
  Constant : Constant  Value=0  OutDataTypeStr=single
  Constant1 : Constant  Value=INS_CONST.g  OutDataTypeStr=single
  Constant2 : Constant  Value=[0;0]  VectorParams1D=off  OutDataTypeStr=single
  Gain : Gain  Gain=INS_CONST.dt  OutDataTypeStr=Inherit: Same as input
  Gain1 : Gain  Gain=-1  OutDataTypeStr=Inherit: Same as input
  Multiply : Product  Multiplication=Matrix(*)
  Mux : Mux  Inputs=3
  Reshape : Reshape  OutputDimensionality=Customize  OutputDimensions=[3,1]
  Selector : Selector  InputPortWidth=3  IndexOptions=Index vector (dialog)  Indices=[3]  OutputSizes=1
  Selector1 : Selector  InputPortWidth=3  IndexOptions=Index vector (dialog)  Indices=[2]  OutputSizes=1
  Selector2 : Selector  InputPortWidth=3  IndexOptions=Index vector (dialog)  Indices=[3]  OutputSizes=1
  Sum : Sum  Inputs=++|
  Switch : Switch  Criteria=u2 > Threshold
  X_Predict : Outport
  wires:
  Rotation_Data/1 -> Bus Selector2/1
  Bus Selector2/1 -> Multiply/1  "<M_OB>"
  Multiply/1 -> Selector/1  "acc_O"
  Bus Selector2/2 -> Multiply/2  "<acc_B_mPs2>"
  X_Prio/1 -> Selector2/1, Sum/1, Selector1/1
  Selector1/1 -> Gain1/1
  Constant/1 -> Mux/3
  Mux/1 -> Reshape/1
  Reshape/1 -> Gain/1
  Add/1 -> Mux/2
  Constant1/1 -> Add/3
  Selector2/1 -> Add/1  "bias_az"
  Gain1/1 -> Mux/1
  Gain/1 -> Sum/2
  Selector/1 -> Add/2
  Assignment/1 -> Switch/3
  Constant2/1 -> Assignment/2
  TF_Data/1 -> Bus Selector/1
  Sum/1 -> Assignment/1, Switch/1
  Bus Selector/1 -> Switch/2  "<h_R_valid>"
  Switch/1 -> X_Predict/1

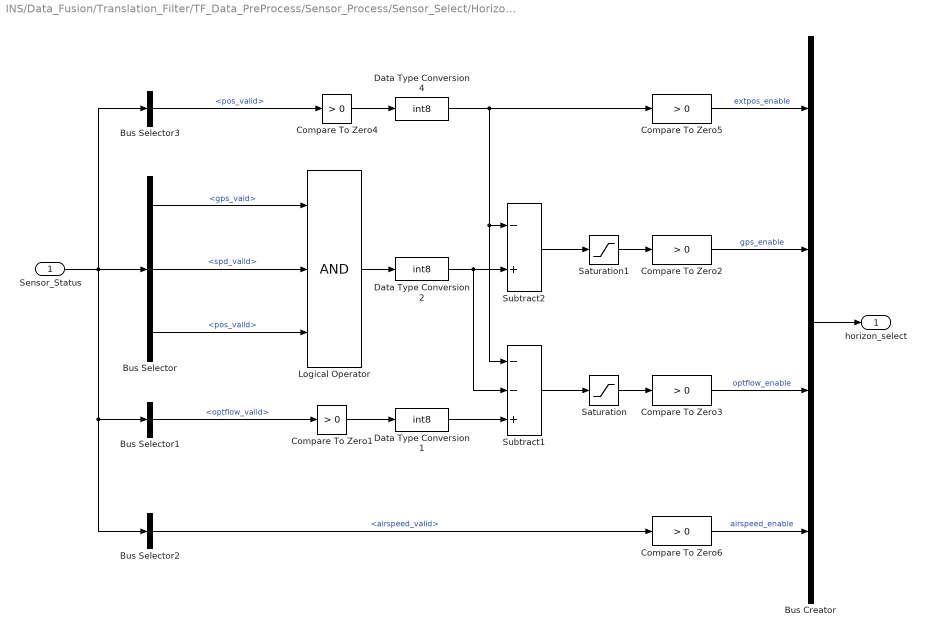
== system INS/Data_Fusion/Translation_Filter/TF_Data_PreProcess/Sensor_Process/Sensor_Select/Horizontal_Sensor_Select ==
  Sensor_Status : Inport
  Bus Creator : BusCreator  Inputs=4
  Bus Selector : BusSelector  OutputSignals=GPS_Status.gps_vaid,GPS_Status.spd_valid,GPS_Status.pos_valid
  Bus Selector1 : BusSelector  OutputSignals=OptFlow_Status.optflow_valid
  Bus Selector2 : BusSelector  OutputSignals=Airspeed_Status.airspeed_valid
  Bus Selector3 : BusSelector  OutputSignals=ExternalPos_Status.pos_valid
  Compare To Zero{1..6} (6 alike) : simulink/Logic and Bit Operations/Compare To Zero  relop=>  OutDataTypeStr=boolean
  Data Type Conversion1 : DataTypeConversion  OutDataTypeStr=int8
  Data Type Conversion2 : DataTypeConversion  OutDataTypeStr=int8
  Data Type Conversion4 : DataTypeConversion  OutDataTypeStr=int8
  Logical Operator : Logic  Inputs=3  AllPortsSameDT=off  OutDataTypeStr=boolean
  Saturation : Saturate  UpperLimit=1  LowerLimit=0
  Saturation1 : Saturate  UpperLimit=1  LowerLimit=0
  Subtract1 : Sum  Inputs=--+
  Subtract2 : Sum  Inputs=-+
  horizon_select : Outport
  wires:
  Bus Selector/1 -> Logical Operator/1  "<gps_vaid>"
  Logical Operator/1 -> Data Type Conversion2/1
  Compare To Zero2/1 -> Bus Creator/2  "gps_enable"
  Bus Creator/1 -> horizon_select/1
  Bus Selector/2 -> Logical Operator/2  "<spd_valid>"
  Bus Selector/3 -> Logical Operator/3  "<pos_valid>"
  Subtract1/1 -> Saturation/1
  Data Type Conversion1/1 -> Subtract1/3
  Bus Selector1/1 -> Compare To Zero1/1  "<optflow_valid>"
  Saturation/1 -> Compare To Zero3/1
  Compare To Zero3/1 -> Bus Creator/3  "optflow_enable"
  Bus Selector3/1 -> Compare To Zero4/1  "<pos_valid>"
  Sensor_Status/1 -> Bus Selector3/1, Bus Selector2/1, Bus Selector1/1, Bus Selector/1
  Compare To Zero5/1 -> Bus Creator/1  "extpos_enable"
  Subtract2/1 -> Saturation1/1
  Data Type Conversion4/1 -> Subtract1/1, Subtract2/1, Compare To Zero5/1
  Data Type Conversion2/1 -> Subtract2/2, Subtract1/2
  Saturation1/1 -> Compare To Zero2/1
  Compare To Zero1/1 -> Data Type Conversion1/1
  Compare To Zero4/1 -> Data Type Conversion4/1
  Bus Selector2/1 -> Compare To Zero6/1  "<airspeed_valid>"
  Compare To Zero6/1 -> Bus Creator/4  "airspeed_enable"

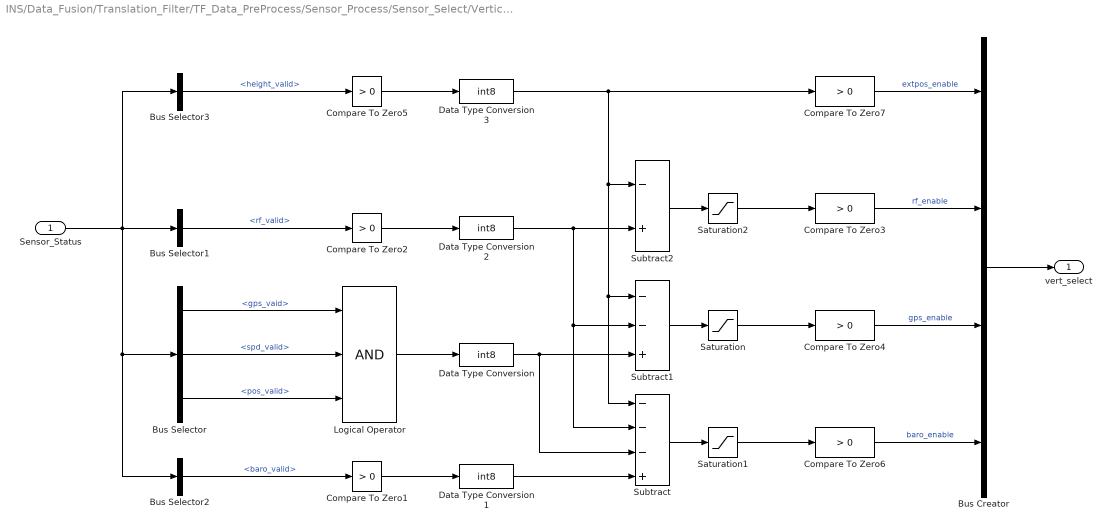
== system INS/Data_Fusion/Translation_Filter/TF_Data_PreProcess/Sensor_Process/Sensor_Select/Vertical_Sensor_Select ==
  Sensor_Status : Inport
  Bus Creator : BusCreator  Inputs=4
  Bus Selector : BusSelector  OutputSignals=GPS_Status.gps_vaid,GPS_Status.spd_valid,GPS_Status.pos_valid
  Bus Selector1 : BusSelector  OutputSignals=Rf_Status.rf_valid
  Bus Selector2 : BusSelector  OutputSignals=Baro_Status.baro_valid
  Bus Selector3 : BusSelector  OutputSignals=ExternalPos_Status.height_valid
  Compare To Zero{1..7} (7 alike) : simulink/Logic and Bit Operations/Compare To Zero  relop=>  OutDataTypeStr=boolean
  Data Type Conversion{,1..3} (4 alike) : DataTypeConversion  OutDataTypeStr=int8
  Logical Operator : Logic  Inputs=3  AllPortsSameDT=off  OutDataTypeStr=boolean
  Saturation : Saturate  UpperLimit=1  LowerLimit=0
  Saturation1 : Saturate  UpperLimit=1  LowerLimit=0
  Saturation2 : Saturate  UpperLimit=1  LowerLimit=0
  Subtract : Sum  Inputs=---+
  Subtract1 : Sum  Inputs=--+
  Subtract2 : Sum  Inputs=-+
  vert_select : Outport
  wires:
  Logical Operator/1 -> Data Type Conversion/1
  Subtract1/1 -> Saturation/1
  Bus Selector/2 -> Logical Operator/2  "<spd_valid>"
  Bus Selector2/1 -> Compare To Zero1/1  "<baro_valid>"
  Compare To Zero1/1 -> Data Type Conversion1/1
  Subtract/1 -> Saturation1/1
  Saturation1/1 -> Compare To Zero6/1
  Data Type Conversion1/1 -> Subtract/4
  Bus Selector/1 -> Logical Operator/1  "<gps_vaid>"
  Bus Selector/3 -> Logical Operator/3  "<pos_valid>"
  Compare To Zero4/1 -> Bus Creator/3  "gps_enable"
  Compare To Zero6/1 -> Bus Creator/4  "baro_enable"
  Bus Creator/1 -> vert_select/1
  Bus Selector1/1 -> Compare To Zero2/1  "<rf_valid>"
  Compare To Zero2/1 -> Data Type Conversion2/1
  Data Type Conversion/1 -> Subtract/3, Subtract1/3
  Data Type Conversion2/1 -> Subtract2/2, Subtract/2, Subtract1/2
  Saturation/1 -> Compare To Zero4/1
  Compare To Zero3/1 -> Bus Creator/2  "rf_enable"
  Sensor_Status/1 -> Bus Selector/1, Bus Selector2/1, Bus Selector3/1, Bus Selector1/1
  Compare To Zero7/1 -> Bus Creator/1  "extpos_enable"
  Data Type Conversion3/1 -> Subtract2/1, Subtract/1, Subtract1/1, Compare To Zero7/1
  Bus Selector3/1 -> Compare To Zero5/1  "<height_valid>"
  Compare To Zero5/1 -> Data Type Conversion3/1
  Subtract2/1 -> Saturation2/1
  Saturation2/1 -> Compare To Zero3/1

== system INS/Data_Fusion/Translation_Filter/TF_Data_PreProcess/Sensor_Process/TF_Sensor_Measures/Airspeed_Meas ==
  Sensor_Data : Inport
  Bus Creator : BusCreator  Inputs=2
  Bus Selector1 : BusSelector  OutputSignals=AirSpeed_Data.timestamp,AirSpeed_Data.IAS
  Signal Copy1 : SignalConversion  OverrideOpt=off
  Signal Copy3 : SignalConversion  OverrideOpt=off
  Airspeed_Meas : Outport
  wires:
  Signal Copy1/1 -> Bus Creator/2  "IAS_mPs"
  Signal Copy3/1 -> Bus Creator/1  "timestamp_ms"
  Bus Selector1/1 -> Signal Copy3/1  "<timestamp>"
  Bus Creator/1 -> Airspeed_Meas/1
  Bus Selector1/2 -> Signal Copy1/1  "<IAS>"
  Sensor_Data/1 -> Bus Selector1/1

== system INS/Data_Fusion/Translation_Filter/TF_Data_PreProcess/Sensor_Process/TF_Sensor_Measures/Barometer_Meas ==
  Sensor_Data : Inport
  Bus Creator : BusCreator  Inputs=3
  Bus Selector1 : BusSelector  OutputSignals=Baro_Data.timestamp,Baro_Data.h_R_m
  Second Order LPF : FMT_Model_Lib/Filter/Second Order LPF  fc=5  zeta=0.707
      settings: SourceProductName=FMT Toolbox
  Signal Copy1 : SignalConversion  OverrideOpt=off
  Signal Copy3 : SignalConversion  OverrideOpt=off
  Baro_Meas : Outport
  wires:
  Sensor_Data/1 -> Bus Selector1/1
  Bus Selector1/2 -> Signal Copy1/1  "<h_R_m>"
  Bus Creator/1 -> Baro_Meas/1
  Bus Selector1/1 -> Signal Copy3/1  "<timestamp>"
  Signal Copy3/1 -> Bus Creator/1  "timestamp_ms"
  Signal Copy1/1 -> Second Order LPF/1, Bus Creator/2  "h_R_m"
  Second Order LPF/1 -> Bus Creator/3  "h_R_filter_m"

== system INS/Data_Fusion/Translation_Filter/TF_Data_PreProcess/Sensor_Process/TF_Sensor_Measures/ExternalPos_Meas ==
  Sensor_Data : Inport
  Rotation_Data : Inport  Port=2
  Bus Creator1 : BusCreator  Inputs=4
  External_Pos_PreProcess : Subsystem
  ExtPos_Meas : Outport
  wires:
  Sensor_Data/1 -> External_Pos_PreProcess/1(Sensor_Data)
  Bus Creator1/1 -> ExtPos_Meas/1
  Rotation_Data/1 -> External_Pos_PreProcess/2(Rotation_Data)
  External_Pos_PreProcess/1(timestamp) -> Bus Creator1/1  "timestamp_ms"
  External_Pos_PreProcess/2(x) -> Bus Creator1/2  "x_O_m"
  External_Pos_PreProcess/3(y) -> Bus Creator1/3  "y_O_m"
  External_Pos_PreProcess/4(h) -> Bus Creator1/4  "h_O_m"

== system INS/Data_Fusion/Translation_Filter/TF_Data_PreProcess/Sensor_Process/TF_Sensor_Measures/GPS_Meas ==
  Sensor_Data : Inport
  Bus Creator : BusCreator  Inputs=14
  Bus Selector : BusSelector  OutputSignals=GPS_Data.dx_dlat,GPS_Data.dy_dlon,GPS_Data.dz_dh,GPS_Data.lat_rad,GPS_Data.lon_rad,GPS_Data.height_m,GPS_Data.vn_mPs,GPS_Data.ve_mPs,GPS_Data.vd_mPs,GPS_Data.timestamp_ms,GPS_Data.spd_quality,GPS_Data.pos_quality
  Constant : Constant  Value=0  OutDataTypeStr=double
  Constant1 : Constant  Value=0  OutDataTypeStr=double
  Signal Copy{,1..11} (12 alike) : SignalConversion  OverrideOpt=off
  GPS_Meas : Outport
  wires:
  Bus Selector/11 -> Signal Copy10/1  "<spd_quality>"
  Signal Copy9/1 -> Bus Creator/10  "timestamp_ms"
  Signal Copy8/1 -> Bus Creator/9  "vd_mPs"
  Signal Copy7/1 -> Bus Creator/8  "ve_mPs"
  Signal Copy6/1 -> Bus Creator/7  "vn_mPs"
  Signal Copy5/1 -> Bus Creator/6  "h_m"
  Signal Copy4/1 -> Bus Creator/5  "lon_rad"
  Signal Copy3/1 -> Bus Creator/4  "lat_rad"
  Signal Copy2/1 -> Bus Creator/3  "dz_dh"
  Signal Copy1/1 -> Bus Creator/2  "dy_dlon"
  Signal Copy/1 -> Bus Creator/1  "dx_dlat"
  Bus Selector/10 -> Signal Copy9/1  "<timestamp_ms>"
  Bus Selector/9 -> Signal Copy8/1  "<vd_mPs>"
  Bus Selector/8 -> Signal Copy7/1  "<ve_mPs>"
  Bus Selector/7 -> Signal Copy6/1  "<vn_mPs>"
  Bus Selector/6 -> Signal Copy5/1  "<height_m>"
  Bus Selector/5 -> Signal Copy4/1  "<lon_rad>"
  Bus Selector/4 -> Signal Copy3/1  "<lat_rad>"
  Bus Selector/3 -> Signal Copy2/1  "<dz_dh>"
  Bus Selector/2 -> Signal Copy1/1  "<dy_dlon>"
  Bus Selector/1 -> Signal Copy/1  "<dx_dlat>"
  Bus Creator/1 -> GPS_Meas/1
  Sensor_Data/1 -> Bus Selector/1
  Bus Selector/12 -> Signal Copy11/1  "<pos_quality>"
  Signal Copy10/1 -> Bus Creator/11  "spd_quality"
  Signal Copy11/1 -> Bus Creator/12  "pos_quality"
  Constant/1 -> Bus Creator/13  "x_m"
  Constant1/1 -> Bus Creator/14  "y_m"

== system INS/Data_Fusion/Translation_Filter/TF_Data_PreProcess/Sensor_Process/TF_Sensor_Measures/OpticalFlow_Meas ==
  Sensor_Data : Inport
  Rotation_Data : Inport  Port=2
  Bus Creator : BusCreator  Inputs=3
  Bus Selector : BusSelector  OutputSignals=M_CO
  Bus Selector1 : BusSelector  OutputSignals=OpticalFlow_Data.timestamp
  Bus Selector2 : BusSelector  OutputSignals=OpticalFlow_Data.vx,OpticalFlow_Data.vy
  Constant : Constant  Value=0  OutDataTypeStr=single
  Multiply : Product  Multiplication=Matrix(*)
  Mux : Mux  Inputs=3
  Selector : Selector  InputPortWidth=3  IndexOptions=Index vector (dialog)  Indices=1  OutputSizes=1
  Selector1 : Selector  InputPortWidth=3  IndexOptions=Index vector (dialog)  Indices=2  OutputSizes=1
  Signal Copy3 : SignalConversion  OverrideOpt=off
  Transpose : Math  Operator=transpose  SaturateOnIntegerOverflow=on
  OptFlow_Meas : Outport
  wires:
  Sensor_Data/1 -> Bus Selector2/1, Bus Selector1/1
  Bus Creator/1 -> OptFlow_Meas/1
  Bus Selector1/1 -> Signal Copy3/1  "<timestamp>"
  Signal Copy3/1 -> Bus Creator/1  "timestamp_ms"
  Rotation_Data/1 -> Bus Selector/1
  Bus Selector/1 -> Transpose/1  "<M_CO>"
  Transpose/1 -> Multiply/1  "M_OC"
  Bus Selector2/1 -> Mux/1  "<vx>"
  Bus Selector2/2 -> Mux/2  "<vy>"
  Constant/1 -> Mux/3
  Mux/1 -> Multiply/2
  Selector/1 -> Bus Creator/2  "vx_O_mPs"
  Multiply/1 -> Selector1/1, Selector/1
  Selector1/1 -> Bus Creator/3  "vy_O_mPs"

== system INS/Data_Fusion/Translation_Filter/TF_Data_PreProcess/Sensor_Process/TF_Sensor_Measures/Rangefinder_Meas ==
  Sensor_Data : Inport
  Bus Creator : BusCreator  Inputs=2
  Bus Selector1 : BusSelector  OutputSignals=Rangefinder_Data.timestamp,Rangefinder_Data.distance
  Signal Copy1 : SignalConversion  OverrideOpt=off
  Signal Copy3 : SignalConversion  OverrideOpt=off
  Rf_Meas : Outport
  wires:
  Signal Copy1/1 -> Bus Creator/2  "h_AGL_m"
  Signal Copy3/1 -> Bus Creator/1  "timestamp_ms"
  Bus Selector1/1 -> Signal Copy3/1  "<timestamp>"
  Bus Creator/1 -> Rf_Meas/1
  Bus Selector1/2 -> Signal Copy1/1  "<distance>"
  Sensor_Data/1 -> Bus Selector1/1

== system INS/Data_Fusion/Translation_Filter/TF_Data_PreProcess/Sensor_Process/TF_Sensor_Status/Airspeed_Status ==
  Sensor_Data : Inport
  Bus Creator : BusCreator  Inputs=1
  Bus Selector : BusSelector  OutputSignals=AirSpeed_Data.valid
  Signal Copy : SignalConversion  OverrideOpt=off
  Airspeed_Status : Outport
  wires:
  Signal Copy/1 -> Bus Creator/1  "airspeed_valid"
  Sensor_Data/1 -> Bus Selector/1
  Bus Creator/1 -> Airspeed_Status/1
  Bus Selector/1 -> Signal Copy/1  "<valid>"

== system INS/Data_Fusion/Translation_Filter/TF_Data_PreProcess/Sensor_Process/TF_Sensor_Status/Barometer_Status ==
  Sensor_Data : Inport
  Bus Creator : BusCreator  Inputs=1
  Bus Selector : BusSelector  OutputSignals=Baro_Data.baro_valid
  Signal Copy : SignalConversion  OverrideOpt=off
  Baro_Status : Outport
  wires:
  Bus Selector/1 -> Signal Copy/1  "<baro_valid>"
  Bus Creator/1 -> Baro_Status/1
  Sensor_Data/1 -> Bus Selector/1
  Signal Copy/1 -> Bus Creator/1  "baro_valid"
